simulink model "CMG_Drive"  (R2024a)
settings: Solver=FixedStepDiscrete  StartTime=0.0  StopTime=8  FixedStep=0.001  RelTol=1e-3
settings Model: Creator=zz  LastModifiedBy=zz

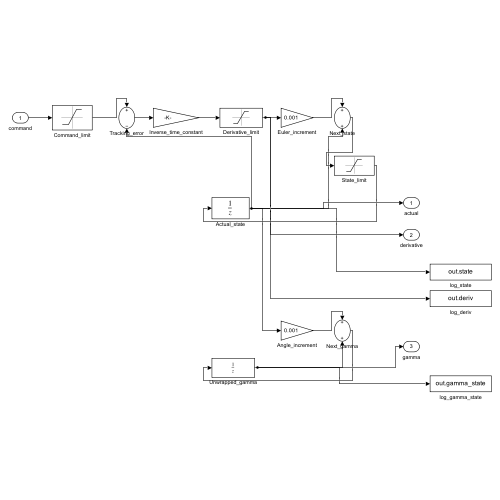
[thumbnail: Simulink's stored preview of the top-level diagram]
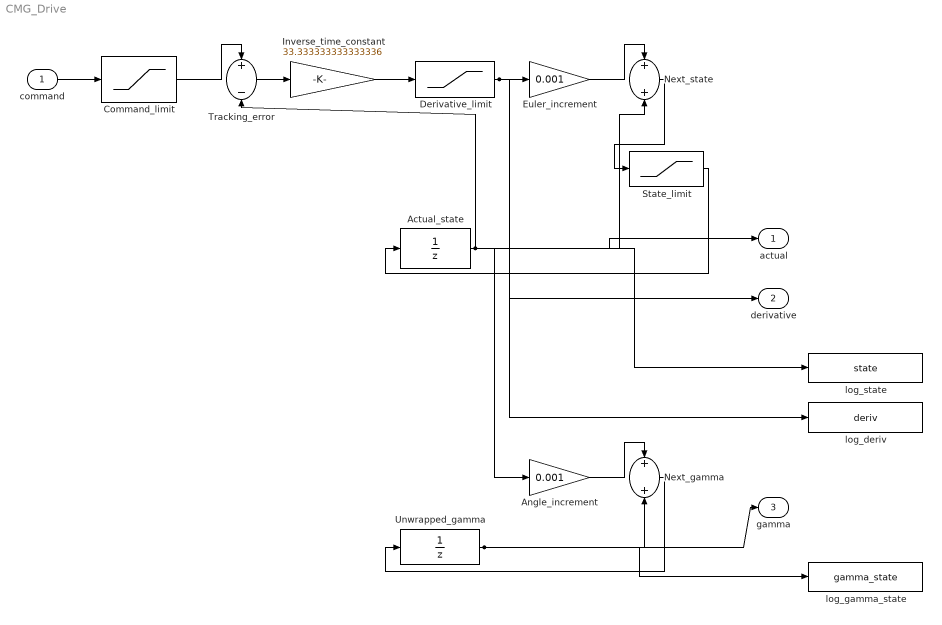
== system CMG_Drive ==
  command : Inport  PortDimensions=4  SampleTime=0.001
  Actual_state : UnitDelay  InitialCondition=[0;0;0;0]  SampleTime=0.001
  Angle_increment : Gain  Gain=0.001
  Command_limit : Saturate  UpperLimit=[1;1;1;1]  LowerLimit=[-1;-1;-1;-1]
  Derivative_limit : Saturate  UpperLimit=[3;3;3;3]  LowerLimit=[-3;-3;-3;-3]
  Euler_increment : Gain  Gain=0.001
  Inverse_time_constant : Gain  Gain=33.333333333333336
  Next_gamma : Sum
  Next_state : Sum
  State_limit : Saturate  UpperLimit=[1;1;1;1]  LowerLimit=[-1;-1;-1;-1]
  Tracking_error : Sum  Inputs=+-
  Unwrapped_gamma : UnitDelay  InitialCondition=zeros(4,1)  SampleTime=0.001
  log_deriv : ToWorkspace  VariableName=deriv  SaveFormat=Timeseries
  log_gamma_state : ToWorkspace  VariableName=gamma_state  SaveFormat=Timeseries
  log_state : ToWorkspace  VariableName=state  SaveFormat=Timeseries
  actual : Outport
  derivative : Outport  Port=2
  gamma : Outport  Port=3
  wires:
  command/1 -> Command_limit/1
  Command_limit/1 -> Tracking_error/1
  Actual_state/1 -> Tracking_error/2, Next_state/2, actual/1, log_state/1, Angle_increment/1
  Tracking_error/1 -> Inverse_time_constant/1
  Inverse_time_constant/1 -> Derivative_limit/1
  Derivative_limit/1 -> Euler_increment/1, derivative/1, log_deriv/1
  Euler_increment/1 -> Next_state/1
  Next_state/1 -> State_limit/1
  State_limit/1 -> Actual_state/1
  Angle_increment/1 -> Next_gamma/1
  Unwrapped_gamma/1 -> Next_gamma/2, gamma/1, log_gamma_state/1
  Next_gamma/1 -> Unwrapped_gamma/1
